simulink library "blocchi_telefono"  (R2023b)
settings: Solver=VariableStepAuto  StartTime=0.0  StopTime=10.0  RelTol=1e-3
undefined symbols (not defined in the file or in its folder): telefono_avvio_automatico
settings Model: Creator=simonefildi  LastModifiedBy=simonefildi
settings ModelReferenceCC: UpdateModelReferenceTargets=IfOutOfDate
settings SFSimCC: SimGPUStackLimitPerThread=51200
settings RTWCC: GPUStackLimitPerThread=51200  GPUComputeCapability=7.5
settings ConfigComp: CovMetricSettings=de  CovBoundaryAbsTol=1.0e-5

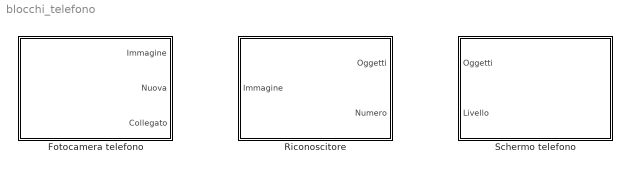
== system blocchi_telefono ==
  Fotocamera telefono : Subsystem  LoadFcn=telefono_avvio_automatico(gcb)  mask(Fotocamera telefono){Altezza=640, Larghezza=480, Passo=0.1, AvvioAutomatico=on}
      mask prompts: Altezza "Altezza immagine (pixel)"; Larghezza "Larghezza immagine (pixel)"; Passo "Ogni quanto leggere una foto (s): 0.1 = 10 foto al secondo"; AvvioAutomatico "Avvio automatico: all'apertura del modello compare il QR code e la simulazione parte da sola quando il telefono invia le foto"
      mask help:
      | Immagini dalla fotocamera del telefono (web app collegata con il QR code).
      | Con Avvio automatico basta aprire il modello: compare il QR code e la simulazione parte da sola quando il telefono comincia a inviare le foto.
      | Immagine: Altezza x Larghezza x 3, uint8. Nuova: 1 se la foto e' appena arrivata. Collegato: 1 se il telefono sta inviando.
      mask Display: port_label('output', 1, 'Immagine'); port_label('output', 2, 'Nuova'); port_label('output', 3, 'Collegato'); disp('Fotocamera\ntelefono')
  Riconoscitore : Subsystem  mask(Riconoscitore){Etichette=, Modello=oggetti, Soglia=0.25, MaxOggetti=10}
      mask prompts: Etichette "Cosa riconoscere (etichette del modello separate da virgola; vuoto = tutte)"; Modello "Modello (oggetti, frutta, bottiglie, ...)"; Soglia "Punteggio minimo (0-1)"; MaxOggetti "Numero massimo di oggetti"
      mask help:
      | Riconosce oggetti con una rete YOLOE (gira in MATLAB, Deep Learning Toolbox).
      | Modello: il nome di una cartella in modelli (oggetti, frutta, bottiglie, ...).
      | Cosa riconoscere: alcune etichette del modello, separate da virgola, es. apple, pear. Vuoto = tutte le etichette del modello.
      | Oggetti: MaxOggetti righe [x y larghezza altezza punteggio classe], righe di zeri se vuote. La classe e' il numero dell'etichetta nell'elenco.
      mask init:
      | IdParametri = parametri_blocco(gcbh, struct('Modello', Modello, 'Etichette', Etichette));
      | if isempty(strtrim(Etichette)), testoBlocco = sprintf('Riconoscitore\n%s: tutto', Modello); else, testoBlocco = sprintf('Riconoscitore\n%s: %s', Modello, Etichette); end
      mask DialogControl ScegliElenco Prompt: Scegli modello e oggetti dall'elenco...
      mask DialogControl ScegliElenco Callback: riconoscitore_scegli(gcb)
      mask Display: port_label('input', 1, 'Immagine'); port_label('output', 1, 'Oggetti'); port_label('output', 2, 'Numero'); disp(testoBlocco)
  Schermo telefono : Subsystem  mask(Schermo telefono){Messaggi=Tutto ok|Attenzione|Pericolo, Colori=verde|giallo|rosso}
      mask prompts: Messaggi "Messaggi (separati da |)"; Colori "Colori (verde, giallo, rosso, grigio, blu o #RRGGBB)"
      mask help:
      | Mostra sul telefono gli Oggetti (riquadri ed elenco).
      | Livello 0: solo cosa si vede. Livello 1, 2, 3...: titolo = Messaggio n. Livello, nel colore n. Livello.
      mask init:
      | IdParametri = parametri_blocco(gcbh, struct('Messaggi', Messaggi, 'Colori', Colori));
      mask Display: port_label('input', 1, 'Oggetti'); port_label('input', 2, 'Livello'); disp('Schermo\ntelefono')

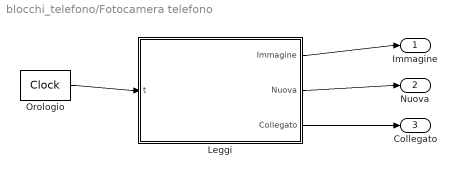
== system blocchi_telefono/Fotocamera telefono ==
  Leggi : MATLAB Function  TreatAsAtomicUnit=on
  Orologio : DigitalClock  SampleTime=Passo
  Immagine : Outport
  Nuova : Outport  Port=2
  Collegato : Outport  Port=3
  wires:
  Orologio/1 -> Leggi/1(t)
  Leggi/1(Immagine) -> Immagine/1
  Leggi/2(Nuova) -> Nuova/1
  Leggi/3(Collegato) -> Collegato/1

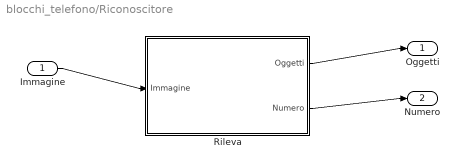
== system blocchi_telefono/Riconoscitore ==
  Immagine : Inport
  Rileva : MATLAB Function  TreatAsAtomicUnit=on
  Oggetti : Outport
  Numero : Outport  Port=2
  wires:
  Immagine/1 -> Rileva/1(Immagine)
  Rileva/1(Oggetti) -> Oggetti/1
  Rileva/2(Numero) -> Numero/1

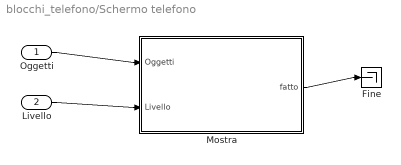
== system blocchi_telefono/Schermo telefono ==
  Oggetti : Inport
  Livello : Inport  Port=2
  Fine : Terminator
  Mostra : MATLAB Function  TreatAsAtomicUnit=on
  wires:
  Oggetti/1 -> Mostra/1(Oggetti)
  Livello/1 -> Mostra/2(Livello)
  Mostra/1(fatto) -> Fine/1

== matlab function blocchi_telefono/Riconoscitore/Rileva ==
  data: Immagine input; Oggetti output; Numero output; IdParametri parameter; Soglia parameter; MaxOggetti parameter
function [Oggetti, Numero] = Rileva(Immagine, IdParametri, Soglia, MaxOggetti)
% Oggetti: una riga per oggetto [x y larghezza altezza punteggio classe].
coder.extrinsic('riconoscitore_simulink');
Oggetti = zeros(MaxOggetti, 6);
Numero = 0;
[Oggetti, Numero] = riconoscitore_simulink(Immagine, IdParametri, Soglia, MaxOggetti);

== matlab function blocchi_telefono/Fotocamera telefono/Leggi ==
  data: t input; Immagine output; Nuova output; Collegato output; Altezza parameter; Larghezza parameter; Passo parameter
function [Immagine, Nuova, Collegato] = Leggi(t, Altezza, Larghezza, Passo) %#ok<INUSD>
% Ultima foto dal telefono, ridimensionata ad Altezza x Larghezza.
coder.extrinsic('telefono_fotocamera');
Immagine = zeros(Altezza, Larghezza, 3, 'uint8');
Nuova = false;
Collegato = false;
[Immagine, Nuova, Collegato] = telefono_fotocamera(Altezza, Larghezza, Passo);

== matlab function blocchi_telefono/Schermo telefono/Mostra ==
  data: Oggetti input; fatto output; Livello input; IdParametri parameter
function fatto = Mostra(Oggetti, Livello, IdParametri)
% Mostra sul telefono gli oggetti e il messaggio scelto da Livello.
coder.extrinsic('telefono_schermo');
telefono_schermo(Oggetti, double(Livello), IdParametri);
fatto = 1;
